simulink model "generator_open_circuit"  (R2021a)
settings: Solver=FixedStepAuto  StartTime=0.0  StopTime=10.0  FixedStep=1e-4  RelTol=1e-3
values from neighbouring files (symbols this model uses):
  p = 5    [generator_parameters.m]
  phi = 0.27    [generator_parameters.m]
libraries: simulink x1, spspowerguiLib x1

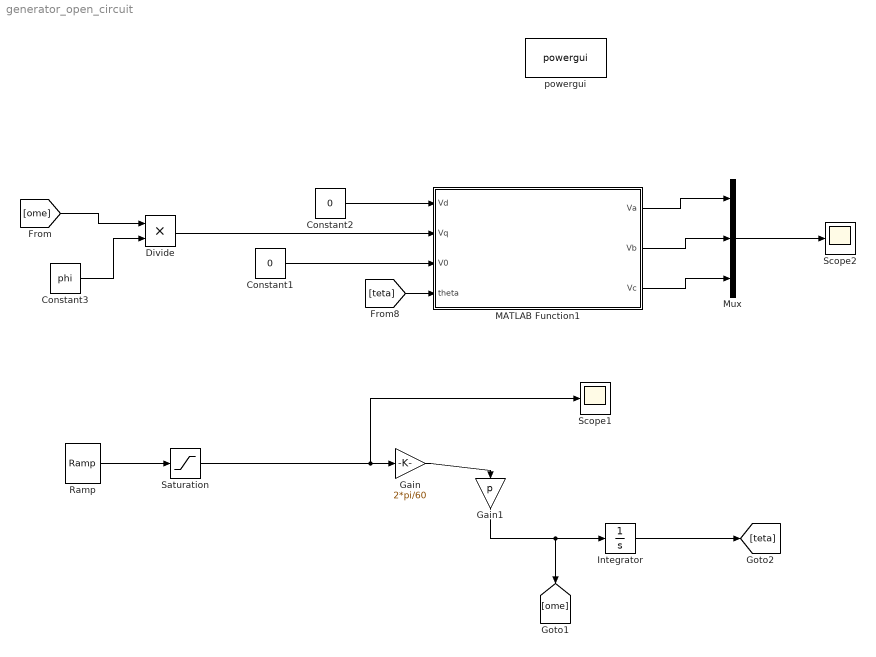
== system generator_open_circuit ==
  Constant1 : Constant  Value=0
  Constant2 : Constant  Value=0
  Constant3 : Constant  Value=phi
  Divide : Product  Inputs=**
  Gain : Gain  Gain=2*pi/60
  Gain1 : Gain  Gain=p
  Integrator : Integrator
  MATLAB Function1 : MATLAB Function  TreatAsAtomicUnit=on
  Mux : Mux  Inputs=3
  Ramp : simulink/Sources/Ramp  slope=1200  start=0  InitialOutput=0
  Saturation : Saturate  UpperLimit=600  LowerLimit=0.5
  Scope1 : Scope
  Scope2 : Scope
  powergui : spspowerguiLib/powergui  Priority=1  SimulationMode=Continuous  SampleTime=50e-6  frequency=60  Iterations=50  frequencyindice=60  Pbase=100e6  ErrMax=1e-4  UnitsV=kV  UnitsW=MW  buscounter=0  FunctionMessages=off  echomessages=off  EnableUseOfTLC=off  CurrentSourceSwitches=off  DisableSnubberDevices=off  DisableRonSwitches=off  DisableVfSwitches=off  DisplayEquations=off  AutomaticDiscreteSolvers=off  SolverType=Tustin/Backward Euler (TBE)  Interpol=off  ExternalGateDelay=off  methode=off  Ts=100  x0status=blocks  SPID=on  SwTol=0  HookPort=off  NonlinearTolerance=1e-4  nMaxIteration=100  ContinueOnMaxIteration=off  RestoreLinks=warning  ResistiveCurrentMeasurement=off  Frange=[0:2:500]  Ylog=off  Xlog=on  ShowGrid=off  save=off  variable=ZData  structure=0  ZoomFFT=off  StartTime=0.0  cycles=1  DisplayStyle=1  fundamental=60  FreqAxis=off  MaxFrequency=1000  frequencyindicesteady=1  RmsSteady=1  display=off
  wires:
  Ramp/1 -> Saturation/1
  Saturation/1 -> Scope1/1, Gain/1
  Gain/1 -> Gain1/1
  Gain1/1 -> Integrator/1, [ome]
  Integrator/1 -> [teta]
  [teta] -> MATLAB Function1/4(theta)
  Divide/1 -> MATLAB Function1/2(Vq)
  Constant1/1 -> MATLAB Function1/3(V0)
  MATLAB Function1/1(Va) -> Mux/1
  MATLAB Function1/2(Vb) -> Mux/2
  MATLAB Function1/3(Vc) -> Mux/3
  Mux/1 -> Scope2/1
  Constant2/1 -> MATLAB Function1/1(Vd)
  [ome] -> Divide/1
  Constant3/1 -> Divide/2

== matlab function generator_open_circuit/MATLAB Function1 ==
  data: Vd input; Va output; Vq input; V0 input; theta input; Vb output; Vc output
function [Va, Vb, Vc] = fcn(Vd, Vq, V0, theta)
    k = sqrt(2/3);
    homopolaire = V0 / sqrt(2); 
    Va = k * (Vd * cos(theta) - Vq * sin(theta) + homopolaire);
    Vb = k * (Vd * cos(theta - 2*pi/3) - Vq * sin(theta - 2*pi/3) + homopolaire);
    Vc = k * (Vd * cos(theta + 2*pi/3) - Vq * sin(theta + 2*pi/3) + homopolaire);
end
